simulink model "tg9"  (R2022a)
settings: Solver=ode15s  StartTime=0.0  StopTime=10  MaxStep=0.01  RelTol=1e-3
InitFcn:
  | mecha_param2
  | control_param0
values from neighbouring files (symbols this model uses):
  b0 = 0    [sim_IMMC.m]
  b1 = 1    [sim_IMMC.m]
  back0 = 0    [sim_IMMC.m]
  back1 = 0    [sim_IMMC.m]
  boff = 0    [sim_IMMC.m]
  bon = 0    [sim_IMMC.m]
  c = 0.05    [mecha_param2.m]
  c_jointstop = 0.3 / (pi/180)    (= 17.1887338539)    [mecha_param2.m]
  calctalus = sqrt((L_foot - (DJ1x_foot))^2 + (H_foot-r_cs)^2)    [mecha_param2.m]
  calctoes = sqrt((H_foot-r_cs)^2 + (DJ1x_foot)^2)    [mecha_param2.m]
  corrD = 0.001    [control_param0.m]
  DG_HAT = 0.35    [mecha_param2.m]
  DG_thigh = 0.28    [mecha_param2.m]
  DJ1x_foot = 0.16-r_cs    (= 0.135)    [mecha_param2.m]
  eref = 0.04    [mecha_param2.m]
  FmaxBFSH = 350    [mecha_param2.m]
  FmaxGAS = 1500    [mecha_param2.m]
  FmaxGLU = 1500    [mecha_param2.m]
  FmaxHAM = 3000    [mecha_param2.m]
  FmaxHFL = 2000    [mecha_param2.m]
  FmaxRF = 1200    [mecha_param2.m]
  FmaxSOL = 4000    [mecha_param2.m]
  FmaxTA = 800    [mecha_param2.m]
  FmaxVAS = 6000    [mecha_param2.m]
  g = 9.81    [mecha_param2.m]
  g0 = 0    [sim_IMMC.m]
  g1 = 0    [sim_IMMC.m]
  H_foot = 0.08    [mecha_param2.m]
  In_HAT = 3    [mecha_param2.m]
  In_shank = 0.05    [mecha_param2.m]
  In_thigh = 0.15    [mecha_param2.m]
  K = 5    [mecha_param2.m]
  knee_thigh = [0 0 -(L_thigh/2)]    [mecha_param2.m]
  Kpress = m_HAT * g / DeltaThRef    (= 104967)    [mecha_param2.m]
  L_foot = 0.2    [mecha_param2.m]
  L_HAT = 0.8    [mecha_param2.m]
  L_shank = 0.46    [mecha_param2.m]
  L_thigh = 0.46    [mecha_param2.m]
  LoHAM = table2array(mt('LoHAM', 1))    [control_param0.m]
  LoHFL = table2array(mt('LoHFL', 1))    [control_param0.m]
  longD = longD - corrD    (= 0.019)    [control_param0.m]
  loptBFSH = 0.12    [mecha_param2.m]
  loptGAS = 0.05    [mecha_param2.m]
  loptGLU = 0.11    [mecha_param2.m]
  loptHAM = 0.10    (= 0.1)    [mecha_param2.m]
  loptHFL = 0.11    [mecha_param2.m]
  loptRF = 0.08    [mecha_param2.m]
  loptSOL = 0.04    [mecha_param2.m]
  loptTA = 0.06    [mecha_param2.m]
  loptVAS = 0.08    [mecha_param2.m]
  LoTA = table2array(mt('LoTA', 1))    [control_param0.m]
  lslackBFSH = 0.10    (= 0.1)    [mecha_param2.m]
  lslackGAS = 0.40    (= 0.4)    [mecha_param2.m]
  lslackGLU = 0.13    [mecha_param2.m]
  lslackHAM = 0.31    [mecha_param2.m]
  lslackHFL = 0.10    (= 0.1)    [mecha_param2.m]
  lslackRF = 0.35    [mecha_param2.m]
  lslackSOL = 0.26    [mecha_param2.m]
  lslackTA = 0.24    [mecha_param2.m]
  lslackVAS = 0.23    [mecha_param2.m]
  m_HAT = 53.5    [mecha_param2.m]
  m_shank = 3.5    [mecha_param2.m]
  m_thigh = 8.5    [mecha_param2.m]
  midD = midD - corrD    (= 0.009)    [control_param0.m]
  N = 1.5    [mecha_param2.m]
  nonoff = 0    [control_param0.m]
  phi_a_low = (70) * (pi / 180)    (= 1.2217304764)    [mecha_param2.m]
  phi_a_up = (130) * (pi / 180)    (= 2.26892802759)    [mecha_param2.m]
  phi_dl = 180    [mecha_param2.m]
  phi_h = 230 * (pi / 180)    (= 4.01425727959)    [mecha_param2.m]
  phi_k = 175 * (pi / 180)    (= 3.05432619099)    [mecha_param2.m]
  phictoes = asind((DJ1y_foot-r_cs)/calctoes)    [mecha_param2.m]
  phimaxGASa = 100*pi/180    (= 1.74532925199)    [mecha_param2.m]
  phimaxGASk = 140*pi/180    (= 2.44346095279)    [mecha_param2.m]
  phimaxRFk = 165*pi/180    (= 2.87979326579)    [mecha_param2.m]
  phimaxSOL = 100*pi/180    (= 1.74532925199)    [mecha_param2.m]
  phimaxTA = 80*pi/180    (= 1.3962634016)    [mecha_param2.m]
  phimaxVAS = 165*pi/180    (= 2.87979326579)    [mecha_param2.m]
  phirefBFSH = 160*pi/180    (= 2.79252680319)    [mecha_param2.m]
  phirefGASa = 80*pi/180    (= 1.3962634016)    [mecha_param2.m]
  phirefGASk = 165*pi/180    (= 2.87979326579)    [mecha_param2.m]
  phirefGLU = 120*pi/180    (= 2.09439510239)    [mecha_param2.m]
  phirefHAMh = 150*pi/180    (= 2.61799387799)    [mecha_param2.m]
  phirefHAMk = 180*pi/180    (= 3.14159265359)    [mecha_param2.m]
  phirefHFL = 160*pi/180    (= 2.79252680319)    [mecha_param2.m]
  phirefRFh = 170*pi/180    (= 2.96705972839)    [mecha_param2.m]
  phirefRFk = 125*pi/180    (= 2.18166156499)    [mecha_param2.m]
  phirefSOL = 90*pi/180    (= 1.57079632679)    [mecha_param2.m]
  phirefTA = 110*pi/180    (= 1.91986217719)    [mecha_param2.m]
  phirefVAS = 120*pi/180    (= 2.09439510239)    [mecha_param2.m]
  phiScaleGASa = acos(rGASamin/rGASamax)/(phiminGASa-phimaxGASa)    [mecha_param2.m]
  phiScaleGASk = acos(rGASkmin/rGASkmax)/(phiminGASk-phimaxGASk)    [mecha_param2.m]
  phiScaleRFk = acos(rRFkmin/rRFkmax)/(phiminRFk-phimaxRFk)    [mecha_param2.m]
  phiScaleSOL = acos(rSOLmin/rSOLmax)/(phiminSOL-phimaxSOL)    [mecha_param2.m]
  phiScaleTA = acos(rTAmin/rTAmax)/(phiminTA-phimaxTA)    [mecha_param2.m]
  phiScaleVAS = acos(rVASmin/rVASmax)/(phiminVAS-phimaxVAS)    [mecha_param2.m]
  r1 = 0    [sim_IMMC.m]
  r_cs = 0.025    [mecha_param2.m]
  rBFSH = 0.04    [mecha_param2.m]
  rGASamax = 0.06    [mecha_param2.m]
  rGASkmax = 0.05    [mecha_param2.m]
  rGLU = 0.08    [mecha_param2.m]
  rHAMh = 0.08    [mecha_param2.m]
  rHAMk = 0.05    [mecha_param2.m]
  rHFL = 0.08    [mecha_param2.m]
  rhoBFSH = 0.7    [mecha_param2.m]
  rhoGASa = 0.7    [mecha_param2.m]
  rhoGASk = 0.7    [mecha_param2.m]
  rhoGLU = 0.5    [mecha_param2.m]
  rhoHAMh = 0.5    [mecha_param2.m]
  rhoHAMk = 0.5    [mecha_param2.m]
  rhoHFL = 0.5    [mecha_param2.m]
  rhoRFh = 0.3    [mecha_param2.m]
  rhoRFk = 0.5    [mecha_param2.m]
  rhoSOL = 0.5    [mecha_param2.m]
  rhoTA = 0.7    [mecha_param2.m]
  rhoVAS = 0.6    [mecha_param2.m]
  rRFh = 0.08    [mecha_param2.m]
  rRFkmax = 0.06    [mecha_param2.m]
  rSOLmax = 0.06    [mecha_param2.m]
  ... (+25 more)
undefined symbols (not defined in the file or in its folder): beta11, beta12, beta13, beta14, beta15, beta16, beta21, beta22, beta23, beta24, beta25, beta26, beta31, beta32, beta33, beta34, beta35, beta36, beta41, beta42, beta43, beta44, beta45, beta46, beta51, beta52, beta53, beta54, beta55, beta56, betab1, betab2, betab3, betab4, betab5, betab6, betap11, betap12, betap13, betap14, betap15, betap16, betap21, betap22, betap23, betap24, betap25, betap26, betap31, betap32, betap33, betap34, betap35, betap36, betap41, betap42, betap43, betap44, betap45, betap46 ... (+102)
libraries: sm_lib x89, simulink x72, nesl_utility x58, simulink_extras x18
(part 2 of 12)

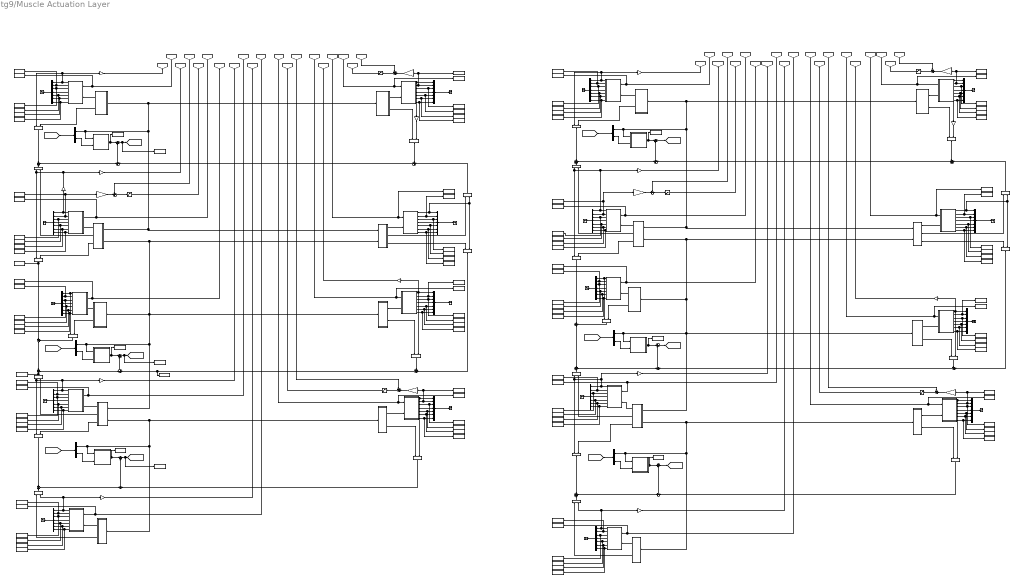
== system tg9/Muscle Actuation Layer ==
  note: L-Lo
  note: Left Hip Joint Mechanics Layer Interface
  note: Right leg - muscular/sensor layer
  note: Muscle Actuator Layer
  note: Left leg - muscular/sensor layer
  note: Left Knee Joint Mechanics Layer Interface
  note: Left Ankle Joint Mechanics Layer Interface
  note: Right Hip Joint Mechanics Layer Interface
  note: Right Knee Joint Mechanics Layer Interface
  note: Right Ankle Joint Mechanics Layer Interface
  note: L-Lo
  note: L-Lo
  note: L-Lo
  note: L-Lo
  note: L-Lo
  Demux{3..8} (6 alike) : Demux  Outputs=2
  Gain : Gain  Gain=1/loptHAM
  Gain1 : Gain  Gain=1/loptHFL
  Gain2 : Gain  Gain=1/loptTA
  Gain3 : Gain  Gain=1/loptHAM
  Gain4 : Gain  Gain=1/loptHFL
  Gain5 : Gain  Gain=1/loptTA
  Gain6 : Gain
  Gain7 : Gain
  Gain9 : Gain
  L Ankle Joint Limit : Subsystem
  L BFSH : Subsystem
  L BFSH Link1 : Subsystem
  L BFSH Link2 : Subsystem
  L GAS : Subsystem
  L GAS Golgi Tendon Organ : Gain
  L GAS Link1 : Subsystem
  L GAS Link2 : Subsystem
  L GLU : Subsystem
  L GLU Golgi Tendon Organ : Gain
  L GLU Link : Subsystem
  L GLU Link1 : Subsystem
  L HAM : Subsystem
  L HAM Golgi Tendon Organ : Gain
  L HAM Link1 : Subsystem
  L HAM Link2 : Subsystem
  L HFL : Subsystem
  L HFL Link1 : Subsystem
  L HFL Link2 : Subsystem
  L Hip Joint Limits : Subsystem
  L Knee Joint Limits : Subsystem
  L RF : Subsystem
  L RF Link1 : Subsystem
  L RF Link2 : Subsystem
  L SOL : Subsystem
  L SOL Golgi Tendon Organ : Gain
  L SOL Link1 : Subsystem
  L SOL Link2 : Subsystem
  L TA : Subsystem
  L TA Link1 : Subsystem
  L TA Link2 : Subsystem
  L VAS : Subsystem
  L VAS Golgi Tendon Organ : Gain
  L VAS Link1 : Subsystem
  L VAS Link2 : Subsystem
  Mux{,1..17} (18 alike) : Mux  Inputs=7
  Product{,1..23} (24 alike) : Product
  R Ankle Joint Limit : Subsystem
  R BFSH : Subsystem
  R GAS : Subsystem
  R GAS Golgi Tendon Organ : Gain
  R GLU : Subsystem
  R GLU Golgi Tendon Organ : Gain
  R HAM Golgi Tendon Organ : Gain
  R HAM1 : Subsystem
  R HFL : Subsystem
  R Hip Joint Limits : Subsystem
  R Knee Joint Limits : Subsystem
  R RF : Subsystem
  R SOL : Subsystem
  R SOL Golgi Tendon Organ : Gain
  R TA : Subsystem
  R VAS : Subsystem
  R VAS Golgi Tendon Organ : Gain
  Saturation{,1..5} (6 alike) : Saturate  UpperLimit=inf  LowerLimit=0  ZeroCross=off
  Sum{,3,6,12,17,20,24,27} (8 alike) : Sum  Inputs=|++
  Sum{1,7,13,21} (4 alike) : Sum  Inputs=+|-
  Sum{9..11,14..15,23} (6 alike) : Sum  Inputs=-+|
  Sum{2,5,8,16,19,22} (6 alike) : Sum  Inputs=+|+
  Sum18 : Sum  Inputs=-|+
  Sum{25..26,28..29} (4 alike) : Sum  Inputs=++|
  Sum4 : Sum  Inputs=-|+
  Terminator{,1..17} (18 alike) : Terminator
  To Workspace : ToWorkspace  VariableName=RHFL_ACT  SampleTime=-1
  To Workspace1 : ToWorkspace  VariableName=RHFL_STIM  SampleTime=-1
  To Workspace10 : ToWorkspace  VariableName=RVAS_STIM  SampleTime=-1
  To Workspace100 : ToWorkspace  VariableName=LRF_FISO  SampleTime=-1
  To Workspace101 : ToWorkspace  VariableName=LRF_LCE  SampleTime=-1
  To Workspace102 : ToWorkspace  VariableName=LBFSH_STIM  SampleTime=-1
  To Workspace103 : ToWorkspace  VariableName=LBFSH_LCE  SampleTime=-1
  To Workspace104 : ToWorkspace  VariableName=LBFSH_ACT  SampleTime=-1
  To Workspace105 : ToWorkspace  VariableName=LBFSH_VCE  SampleTime=-1
  To Workspace106 : ToWorkspace  VariableName=LBFSH_FCE  SampleTime=-1
  To Workspace107 : ToWorkspace  VariableName=LBFSH_FISO  SampleTime=-1
  To Workspace108 : ToWorkspace  VariableName=RBFSH_STIM  SampleTime=-1
  To Workspace109 : ToWorkspace  VariableName=RBFSH_LCE  SampleTime=-1
  To Workspace11 : ToWorkspace  VariableName=RVAS_LCE  SampleTime=-1
  To Workspace110 : ToWorkspace  VariableName=RBFSH_ACT  SampleTime=-1
  To Workspace111 : ToWorkspace  VariableName=RBFSH_VCE  SampleTime=-1
  To Workspace112 : ToWorkspace  VariableName=RBFSH_FCE  SampleTime=-1
  To Workspace113 : ToWorkspace  VariableName=RBFSH_FISO  SampleTime=-1
  To Workspace114 : ToWorkspace  VariableName=RRF_FISO  SampleTime=-1
  To Workspace115 : ToWorkspace  VariableName=RRF_LCE  SampleTime=-1
  To Workspace116 : ToWorkspace  VariableName=RRF_ACT  SampleTime=-1
  To Workspace117 : ToWorkspace  VariableName=RRF_STIM  SampleTime=-1
  To Workspace118 : ToWorkspace  VariableName=RRF_VCE  SampleTime=-1
  To Workspace119 : ToWorkspace  VariableName=RRF_FCE  SampleTime=-1
  To Workspace12 : ToWorkspace  VariableName=RTA_STIM  SampleTime=-1
  To Workspace13 : ToWorkspace  VariableName=RTA_LCE  SampleTime=-1
  To Workspace14 : ToWorkspace  VariableName=RTA_ACT  SampleTime=-1
  To Workspace15 : ToWorkspace  VariableName=RTA_VCE  SampleTime=-1
  To Workspace16 : ToWorkspace  VariableName=RTA_FCE  SampleTime=-1
  To Workspace17 : ToWorkspace  VariableName=RTA_FISO  SampleTime=-1
  To Workspace18 : ToWorkspace  VariableName=RGAS_STIM  SampleTime=-1
  To Workspace19 : ToWorkspace  VariableName=RGAS_LCE  SampleTime=-1
  To Workspace2 : ToWorkspace  VariableName=RHFL_VCE  SampleTime=-1
  To Workspace20 : ToWorkspace  VariableName=RGAS_ACT  SampleTime=-1
  To Workspace21 : ToWorkspace  VariableName=RGAS_VCE  SampleTime=-1
  To Workspace22 : ToWorkspace  VariableName=RGAS_FCE  SampleTime=-1
  To Workspace23 : ToWorkspace  VariableName=RGAS_FISO  SampleTime=-1
  To Workspace24 : ToWorkspace  VariableName=RSOL_STIM  SampleTime=-1
  To Workspace25 : ToWorkspace  VariableName=RSOL_LCE  SampleTime=-1
  To Workspace26 : ToWorkspace  VariableName=RSOL_ACT  SampleTime=-1
  To Workspace27 : ToWorkspace  VariableName=RSOL_VCE  SampleTime=-1
  To Workspace28 : ToWorkspace  VariableName=RSOL_FCE  SampleTime=-1
  To Workspace29 : ToWorkspace  VariableName=RSOL_FISO  SampleTime=-1
  To Workspace3 : ToWorkspace  VariableName=RHFL_FCE  SampleTime=-1
  To Workspace30 : ToWorkspace  VariableName=RHAM_STIM  SampleTime=-1
  To Workspace31 : ToWorkspace  VariableName=RHAM_LCE  SampleTime=-1
  To Workspace32 : ToWorkspace  VariableName=RHAM_ACT  SampleTime=-1
  To Workspace33 : ToWorkspace  VariableName=RHAM_VCE  SampleTime=-1
  To Workspace34 : ToWorkspace  VariableName=RHAM_FCE  SampleTime=-1
  To Workspace35 : ToWorkspace  VariableName=RHAM_FISO  SampleTime=-1
  To Workspace36 : ToWorkspace  VariableName=RGLU_STIM  SampleTime=-1
  To Workspace37 : ToWorkspace  VariableName=RGLU_LCE  SampleTime=-1
  To Workspace38 : ToWorkspace  VariableName=RGLU_ACT  SampleTime=-1
  To Workspace39 : ToWorkspace  VariableName=RGLU_VCE  SampleTime=-1
  To Workspace4 : ToWorkspace  VariableName=RHFL_FISO  SampleTime=-1
  To Workspace40 : ToWorkspace  VariableName=RGLU_FCE  SampleTime=-1
  To Workspace41 : ToWorkspace  VariableName=RGLU_FISO  SampleTime=-1
  To Workspace42 : ToWorkspace  VariableName=LHFL_ACT  SampleTime=-1
  To Workspace43 : ToWorkspace  VariableName=LHFL_STIM  SampleTime=-1
  To Workspace44 : ToWorkspace  VariableName=LHFL_VCE  SampleTime=-1
  To Workspace45 : ToWorkspace  VariableName=LHFL_FCE  SampleTime=-1
  To Workspace46 : ToWorkspace  VariableName=LHFL_FISO  SampleTime=-1
  To Workspace47 : ToWorkspace  VariableName=LHFL_LCE  SampleTime=-1
  To Workspace48 : ToWorkspace  VariableName=LVAS_ACT  SampleTime=-1
  To Workspace49 : ToWorkspace  VariableName=LVAS_STIM  SampleTime=-1
  To Workspace5 : ToWorkspace  VariableName=RHFL_LCE  SampleTime=-1
  To Workspace50 : ToWorkspace  VariableName=LVAS_VCE  SampleTime=-1
  To Workspace51 : ToWorkspace  VariableName=LVAS_FCE  SampleTime=-1
  To Workspace52 : ToWorkspace  VariableName=LVAS_FISO  SampleTime=-1
  To Workspace53 : ToWorkspace  VariableName=LVAS_LCE  SampleTime=-1
  To Workspace54 : ToWorkspace  VariableName=LTA_ACT  SampleTime=-1
  To Workspace55 : ToWorkspace  VariableName=LTA_STIM  SampleTime=-1
  To Workspace56 : ToWorkspace  VariableName=LTA_VCE  SampleTime=-1
  To Workspace57 : ToWorkspace  VariableName=LTA_FCE  SampleTime=-1
  To Workspace58 : ToWorkspace  VariableName=LTA_FISO  SampleTime=-1
  To Workspace59 : ToWorkspace  VariableName=LTA_LCE  SampleTime=-1
  To Workspace6 : ToWorkspace  VariableName=RVAS_ACT  SampleTime=-1
  To Workspace60 : ToWorkspace  VariableName=LGLU_STIM  SampleTime=-1
  To Workspace61 : ToWorkspace  VariableName=LGLU_LCE  SampleTime=-1
  To Workspace62 : ToWorkspace  VariableName=LGLU_ACT  SampleTime=-1
  To Workspace63 : ToWorkspace  VariableName=LGLU_VCE  SampleTime=-1
  To Workspace64 : ToWorkspace  VariableName=LGLU_FCE  SampleTime=-1
  To Workspace65 : ToWorkspace  VariableName=LGLU_FISO  SampleTime=-1
  To Workspace66 : ToWorkspace  VariableName=LHAM_STIM  SampleTime=-1
  To Workspace67 : ToWorkspace  VariableName=LHAM_LCE  SampleTime=-1
  To Workspace68 : ToWorkspace  VariableName=LHAM_ACT  SampleTime=-1
  To Workspace69 : ToWorkspace  VariableName=LHAM_VCE  SampleTime=-1
  To Workspace7 : ToWorkspace  VariableName=RVAS_VCE  SampleTime=-1
  To Workspace70 : ToWorkspace  VariableName=LHAM_FCE  SampleTime=-1
  To Workspace71 : ToWorkspace  VariableName=LHAM_FISO  SampleTime=-1
  To Workspace72 : ToWorkspace  VariableName=LGAS_STIM  SampleTime=-1
  To Workspace73 : ToWorkspace  VariableName=LGAS_LCE  SampleTime=-1
  To Workspace74 : ToWorkspace  VariableName=LGAS_ACT  SampleTime=-1
  To Workspace75 : ToWorkspace  VariableName=LGAS_VCE  SampleTime=-1
  To Workspace76 : ToWorkspace  VariableName=LGAS_FCE  SampleTime=-1
  To Workspace77 : ToWorkspace  VariableName=LGAS_FISO  SampleTime=-1
  To Workspace78 : ToWorkspace  VariableName=LSOL_STIM  SampleTime=-1
  To Workspace79 : ToWorkspace  VariableName=LSOL_LCE  SampleTime=-1
  To Workspace8 : ToWorkspace  VariableName=RVAS_FCE  SampleTime=-1
  To Workspace80 : ToWorkspace  VariableName=LSOL_ACT  SampleTime=-1
  To Workspace81 : ToWorkspace  VariableName=LSOL_VCE  SampleTime=-1
  To Workspace82 : ToWorkspace  VariableName=LSOL_FCE  SampleTime=-1
  To Workspace83 : ToWorkspace  VariableName=LSOL_FISO  SampleTime=-1
  To Workspace84 : ToWorkspace  VariableName=painLhip  SampleTime=-1
  To Workspace85 : ToWorkspace  VariableName=painLknee  SampleTime=-1
  To Workspace86 : ToWorkspace  VariableName=painLankle  SampleTime=-1
  To Workspace87 : ToWorkspace  VariableName=painRankle  SampleTime=-1
  To Workspace88 : ToWorkspace  VariableName=painRknee  SampleTime=-1
  To Workspace89 : ToWorkspace  VariableName=painRhip  SampleTime=-1
  To Workspace9 : ToWorkspace  VariableName=RVAS_FISO  SampleTime=-1
  To Workspace90 : ToWorkspace  VariableName=LhipT  SampleTime=-1
  To Workspace91 : ToWorkspace  VariableName=LkneeT  SampleTime=-1
  To Workspace92 : ToWorkspace  VariableName=LankleT  SampleTime=-1
  To Workspace93 : ToWorkspace  VariableName=VASf  SampleTime=-1
  To Workspace94 : ToWorkspace  VariableName=HAMf  SampleTime=-1
  To Workspace95 : ToWorkspace  VariableName=GASf  SampleTime=-1
  To Workspace96 : ToWorkspace  VariableName=LRF_ACT  SampleTime=-1
  To Workspace97 : ToWorkspace  VariableName=LRF_STIM  SampleTime=-1
  To Workspace98 : ToWorkspace  VariableName=LRF_VCE  SampleTime=-1
  To Workspace99 : ToWorkspace  VariableName=LRF_FCE  SampleTime=-1
  tag scope: LGASgolgi=global, LGLUgolgi=global, LHAMgolgi=global, LHAMspindle=global, LHFLspindle=global, LSOLgolgi=global, LTAspindle=global, LVASgolgi=global, LankleM=global, LhipM=global, LkneeM=global, RGASgolgi=global, RGLUgolgi=global, RHAMgolgi=global, RHAMspindle=global, RHFLspindle=global, RSOLgolgi=global, RTAspindle=global, RVASgolgi=global, RankleM=global, RhipM=global, RkneeM=global
  wires:
  Demux3/1 -> L Hip Joint Limits/1(phi hip [rad]), L GLU Link/1(phi34 [rad]), L HFL Link1/1(phi34 [rad]), L HAM Link2/1(phi34 [rad]), L RF Link1/1(phi34 [rad])
  Demux3/2 -> L Hip Joint Limits/2(dphi hip [rad/s])
  [LHipBMLMAL] -> Demux3/1
  Demux4/1 -> L GAS Link1/1(phi23 [rad]), L BFSH Link1/1(phi23 [rad]), L VAS Link1/1(phi23 [rad]), L HAM Link2/2(phi23 [rad]), L RF Link1/2(phi23 [rad]), L Knee Joint Limits/1(phi [rad])
  [LKneeBMLMAL] -> Demux4/1
  Demux4/2 -> L Knee Joint Limits/2(dphi [rad/s])
  Demux5/2 -> L Ankle Joint Limit/2(dphi [rad/s])
  Demux5/1 -> L SOL Link1/1(phi12 [rad]), L GAS Link1/2(phi12 [rad]), L TA Link1/1(phi12 [rad]), L Ankle Joint Limit/1(phi [rad])
  [LAnkleBMLMAL] -> Demux5/1
  L Hip Joint Limits/1(M_stop [Nm]) -> To Workspace84/1, Sum/1
  Sum/1 -> To Workspace90/1, [LhipM]
  Sum1/1 -> Sum/2
  Sum2/1 -> Sum1/1
  Sum3/1 -> To Workspace91/1, [LkneeM]
  Sum4/1 -> Sum3/2
  Sum5/1 -> Sum4/1
  Sum6/1 -> To Workspace92/1, [LankleM]
  L Ankle Joint Limit/1(M_stop [Nm]) -> To Workspace86/1, Sum6/1
  Sum8/1 -> Sum7/1
  Sum7/1 -> Sum6/2
  [LGLUstim] -> To Workspace60/1, L GLU/1(STIM)
  L GLU Link/1(lmtu [m]) -> L GLU/2(lmtu [m])
  L GLU/1(Fmtc) -> Mux/1, L GLU Golgi Tendon Organ/1, Product/1
  L GLU/2(Lce) -> To Workspace61/1, Mux/2
  L GLU/4(lse) -> Mux/4
  L GLU/5(A) -> To Workspace62/1, Mux/5
  Mux/1 -> Terminator/1
  Mux1/1 -> Terminator7/1
  L HFL/4(lse) -> Mux1/4
  L HFL/2(Lce) -> Mux1/2, To Workspace47/1, Gain1/1
  L HFL/5(A) -> Mux1/5, To Workspace42/1
  L HFL/1(Fmtc) -> Gain6/1, Mux1/1
  L HFL Link1/1(lmtu [m]) -> L HFL/2(lmtu [m])
  L HFL/3(Vce) -> To Workspace44/1, Mux1/3
  [LHFLstim] -> To Workspace43/1, L HFL/1(STIM)
  L VAS/4(lse) -> Mux2/4
  L VAS/1(Fmtc) -> Mux2/1, Product7/2, L VAS Golgi Tendon Organ/1
  L VAS/2(Lce) -> To Workspace53/1, Mux2/2
  L VAS/5(A) -> To Workspace48/1, Mux2/5
  [LVASstim] -> To Workspace49/1, L VAS/1(STIM)
  Mux2/1 -> Terminator1/1
  L HAM/4(lse) -> Mux3/4
  L HAM/1(Fmtc) -> Mux3/1, Gain9/1
  L HAM/2(Lce) -> Mux3/2, Gain/1, To Workspace67/1
  L HAM/5(A) -> Mux3/5, To Workspace68/1
  [LHAMstim] -> To Workspace66/1, L HAM/1(STIM)
  L HAM/3(Vce) -> To Workspace69/1, Mux3/3
  Mux3/1 -> Terminator8/1
  L HAM Link2/1(lmtu [m]) -> L HAM/2(lmtu [m])
  L VAS Link1/1(lmtu [m]) -> L VAS/2(lmtu [m])
  L GAS/4(lse) -> Mux4/4
  L GAS/1(Fmtc) -> Mux4/1, L GAS Golgi Tendon Organ/1, Product4/1, Product3/1
  L GAS/2(Lce) -> To Workspace73/1, Mux4/2
  L GAS/5(A) -> To Workspace74/1, Mux4/5
  L GAS/3(Vce) -> To Workspace75/1, Mux4/3
  Mux4/1 -> Terminator2/1
  L GAS Link1/1(lmtu [m]) -> L GAS/2(lmtu [m])
  L TA Link1/1(lmtc [m]) -> L TA/2(lmtu [m])
  L TA/4(lse) -> Mux5/4
  L TA/1(Fmtc) -> Product6/2, Mux5/1
  L TA/2(Lce) -> Mux5/2, Gain2/1, To Workspace59/1
  L TA/5(A) -> To Workspace54/1, Mux5/5
  [LTAstim] -> To Workspace55/1, L TA/1(STIM)
  L TA/3(Vce) -> To Workspace56/1, Mux5/3
  Mux5/1 -> Terminator3/1
  L SOL/4(lse) -> Mux6/4
  L SOL/1(Fmtc) -> Mux6/1, L SOL Golgi Tendon Organ/1, Product5/2
  L SOL/2(Lce) -> To Workspace79/1, Mux6/2
  L SOL/5(A) -> To Workspace80/1, Mux6/5
  L SOL/3(Vce) -> To Workspace81/1, Mux6/3
  Mux6/1 -> Terminator4/1
  L SOL Link1/1(lmtc [m]) -> L SOL/2(lmtu [m])
  L GLU Link/2(lever [m]) -> Product/2
  Product/1 -> Sum2/1
  Product1/1 -> Sum2/2
  L HAM Link2/2(lever34 [m]) -> Product1/2
  L HAM Link2/3(lever23 [m]) -> Product2/2
  Sum24/1 -> Sum5/1
  Product3/1 -> To Workspace95/1, Sum5/2
  L GAS Link1/2(lever23 [m]) -> Product3/2
  L GAS Link1/3(lever12 [m]) -> Product4/2
  Product4/1 -> Sum8/1
  Product5/1 -> Sum8/2
  L SOL Link1/2(lever [m]) -> Product5/1
  L TA Link1/2(lever [m]) -> Product6/1
  Product6/1 -> Sum7/2
  Sum25/1 -> To Workspace93/1, Sum4/2
  L VAS Link1/2(lever [m]) -> Product7/1
  L VAS/3(Vce) -> To Workspace50/1, Mux2/3
  L HFL Link1/2(lever [m]) -> Product8/1
  Sum26/1 -> Sum1/2
  L GLU Golgi Tendon Organ/1 -> [LGLUgolgi]
  L HAM Golgi Tendon Organ/1 -> [LHAMgolgi]
  L SOL Golgi Tendon Organ/1 -> [LSOLgolgi]
  L GAS Golgi Tendon Organ/1 -> [LGASgolgi]
  Gain/1 -> Sum9/2
  Sum9/1 -> Saturation/1
  Gain1/1 -> Sum10/2
  Sum10/1 -> Saturation1/1
  Gain2/1 -> Sum11/2
  Sum11/1 -> Saturation2/1
  L VAS Golgi Tendon Organ/1 -> [LVASgolgi]
  Saturation/1 -> [LHAMspindle]
  [LyHAM] -> Sum9/1
  [LGASstim] -> To Workspace72/1, L GAS/1(STIM)
  [LSOLstim] -> To Workspace78/1, L SOL/1(STIM)
  [LyTA] -> Sum11/1
  [LyHFL] -> Sum10/1
  Saturation2/1 -> [LTAspindle]
  Saturation1/1 -> [LHFLspindle]
  Demux8/1 -> R Ankle Joint Limit/1(phi [rad]), L SOL Link2/1(phi12 [rad]), L TA Link2/1(phi12 [rad]), L GAS Link2/2(phi12 [rad])
  Saturation4/1 -> [RHFLspindle]
  Product11/1 -> Sum27/1
  Mux7/1 -> Terminator5/1
  L GLU Link1/2(lever [m]) -> Product9/2
  L SOL Link2/2(lever [m]) -> Product14/1
  Mux9/1 -> Terminator6/1
  Sum17/1 -> [RkneeM]
  Gain4/1 -> Sum14/2
  R VAS/1(Fmtc) -> R VAS Golgi Tendon Organ/1, Product16/2, Mux9/1
  L TA Link2/1(lmtc [m]) -> R TA/2(lmtu [m])
  R GAS Golgi Tendon Organ/1 -> [RGASgolgi]
  R VAS/3(Vce) -> To Workspace7/1, Mux9/3
  Saturation5/1 -> [RTAspindle]
  R SOL/4(lse) -> Mux13/4
  R VAS Golgi Tendon Organ/1 -> [RVASgolgi]
  [RyHFL] -> Sum14/1
  Gain3/1 -> Sum23/2
  Sum16/1 -> Sum13/1
  [RGASstim] -> R GAS/1(STIM), To Workspace18/1
  Sum18/1 -> Sum17/2
  R TA/2(Lce) -> Gain5/1, To Workspace13/1, Mux12/2
  Sum15/1 -> Saturation5/1
  R SOL Golgi Tendon Organ/1 -> [RSOLgolgi]
  L HAM Link1/2(lever34 [m]) -> Product10/2
  Sum28/1 -> Sum18/2
  [RyTA] -> Sum15/1
  [RyHAM] -> Sum23/1
  R Ankle Joint Limit/1(M_stop [Nm]) -> To Workspace87/1, Sum20/1
  R VAS/2(Lce) -> Mux9/2, To Workspace11/1
  R GLU Golgi Tendon Organ/1 -> [RGLUgolgi]
  L HFL Link2/2(lever [m]) -> Product17/1
  R HFL/3(Vce [m/s]) -> To Workspace2/1, Mux8/3
  Mux11/1 -> Terminator9/1
  R VAS/5(A) -> To Workspace6/1, Mux9/5
  Saturation3/1 -> [RHAMspindle]
  Sum13/1 -> Sum12/2
  Sum14/1 -> Saturation4/1
  Sum23/1 -> Saturation3/1
  Sum29/1 -> Sum13/2
  Sum20/1 -> [RankleM]
  Product13/1 -> Sum22/1
  R HAM1/3(Vce) -> Mux10/3, To Workspace33/1
  Product12/1 -> Sum19/2
  L HAM Link1/3(lever23 [m]) -> Product11/2
  L VAS Link2/1(lmtu [m]) -> R VAS/2(lmtu [m])
  R GAS/5(A) -> To Workspace20/1, Mux11/5
  L GAS Link2/2(lever23 [m]) -> Product12/2
  Product14/1 -> Sum22/2
  Product15/1 -> Sum21/2
  L HFL Link2/1(lmtu [m]) -> R HFL/2(lmtu [m])
  L GAS Link2/3(lever12 [m]) -> Product13/2
  L TA Link2/2(lever [m]) -> Product15/1
  R GAS/4(lse) -> Mux11/4
  Product10/1 -> Sum16/2
  [RAnkleBMLMAL] -> Demux8/1
  Product9/1 -> Sum16/1
  Mux12/1 -> Terminator10/1
  L SOL Link2/1(lmtc [m]) -> R SOL/2(lmtu [m])
  Mux13/1 -> Terminator11/1
  R GAS/1(Fmtc) -> Mux11/1, R GAS Golgi Tendon Organ/1, Product12/1, Product13/1
  R GAS/2(Lce) -> To Workspace19/1, Mux11/2
  R VAS/4(lse) -> Mux9/4
  [RHAMstim] -> To Workspace30/1, R HAM1/1(STIM)
  [RHFLstim] -> To Workspace1/1, R HFL/1(STIM)
  R HAM1/2(Lce) -> Mux10/2, To Workspace31/1, Gain3/1
  [RTAstim] -> To Workspace12/1, R TA/1(STIM)
  L GAS Link2/1(lmtu [m]) -> R GAS/2(lmtu [m])
  R TA/3(Vce) -> To Workspace15/1, Mux12/3
  R HAM1/5(A) -> To Workspace32/1, Mux10/5
  R TA/5(A) -> To Workspace14/1, Mux12/5
  R TA/4(lse) -> Mux12/4
  Sum21/1 -> Sum20/2
  R HFL/4(lse [m]) -> Mux8/4
  R HAM1/4(lse) -> Mux10/4
  R GLU/4(lse) -> Mux7/4
  R GLU/3(Vce) -> To Workspace39/1, Mux7/3
  [RGLUstim] -> To Workspace36/1, R GLU/1(STIM)
  L VAS Link2/2(lever [m]) -> Product16/1
  Mux10/1 -> Terminator13/1
  Mux8/1 -> Terminator12/1
  Gain5/1 -> Sum15/2
  R HAM Golgi Tendon Organ/1 -> [RHAMgolgi]
  R GLU/5(A) -> To Workspace38/1, Mux7/5
  R GAS/3(Vce) -> To Workspace21/1, Mux11/3
  [RHipBMLMAL] -> Demux6/1
  R TA/1(Fmtc) -> Product15/2, Mux12/1
  R Knee Joint Limits/1(M_stop [Nm]) -> To Workspace88/1, Sum17/1
  [RKneeBMLMAL] -> Demux7/1
  [RSOLstim] -> To Workspace24/1, R SOL/1(STIM)
  R GLU/2(Lce) -> To Workspace37/1, Mux7/2
  R HFL/2(Lce [m]) -> To Workspace5/1, Gain4/1, Mux8/2
  Sum19/1 -> Sum18/1
  L HAM Link1/1(lmtu [m]) -> R HAM1/2(lmtu [m])
  L GLU Link1/1(lmtu [m]) -> R GLU/2(lmtu [m])
  R Hip Joint Limits/1(M_stop [Nm]) -> To Workspace89/1, Sum12/1
  Demux8/2 -> R Ankle Joint Limit/2(dphi [rad/s])
  R HAM1/1(Fmtc) -> Mux10/1, Product10/1, Product11/1, R HAM Golgi Tendon Organ/1
  R GLU/1(Fmtc) -> Mux7/1, R GLU Golgi Tendon Organ/1, Product9/1
  [RVASstim] -> To Workspace10/1, R VAS/1(STIM)
  Sum12/1 -> [RhipM]
  Demux7/2 -> R Knee Joint Limits/2(dphi [rad/s])
  Sum22/1 -> Sum21/1
  Demux6/2 -> R Hip Joint Limits/2(dphi [rad/s])
  Gain6/1 -> Product8/2
  Gain7/1 -> Product17/2
  Gain9/1 -> Product1/1, Product2/1, L HAM Golgi Tendon Organ/1
  R HFL/5(A) -> To Workspace/1, Mux8/5
  R HFL/1(Fmtc [N]) -> Gain7/1, Mux8/1
  R HFL/6(Fce [N]) -> To Workspace3/1, Mux8/6
  R HFL/7(fse [Fmax]) -> To Workspace4/1, Mux8/7
  R VAS/6(fce [Fmax]) -> To Workspace8/1, Mux9/6
  R VAS/7(fse [Fmax]) -> To Workspace9/1, Mux9/7
  R TA/6(fce [Fmax]) -> To Workspace16/1, Mux12/6
  R TA/7(fse [Fmax]) -> To Workspace17/1, Mux12/7
  R GAS/6(fce [Fmax]) -> To Workspace22/1, Mux11/6
  R GAS/7(fse [Fmax]) -> Mux11/7, To Workspace23/1
  R SOL/7("fse [Fmax}") -> To Workspace29/1, Mux13/7
  R SOL/6("fce [Fmax}") -> To Workspace28/1, Mux13/6
  R SOL/5(A) -> To Workspace26/1, Mux13/5
  R SOL/1(Fmtc) -> Mux13/1, R SOL Golgi Tendon Organ/1, Product14/2
  R SOL/3(Vce) -> To Workspace27/1, Mux13/3
  R SOL/2(Lce) -> Mux13/2, To Workspace25/1
  R HAM1/6(fce [Fmax]) -> To Workspace34/1, Mux10/6
  R HAM1/7(fse [Fmax]) -> To Workspace35/1, Mux10/7
  R GLU/6(fce [Fmax]) -> To Workspace40/1, Mux7/6
  R GLU/7(fse [Fmax]) -> To Workspace41/1, Mux7/7
  L SOL/6(fce [Fmax]) -> To Workspace82/1, Mux6/6
  L SOL/7("fse [Fmax}") -> To Workspace83/1, Mux6/7
  L GAS/6(fce [Fmax]) -> To Workspace76/1, Mux4/6
  L GAS/7("fse [Fmax}") -> To Workspace77/1, Mux4/7
  L HAM/6(fce [Fmax]) -> Mux3/6, To Workspace70/1
  L HAM/7("fse [Fmax}") -> To Workspace71/1, Mux3/7
  L GLU/6(fce [Fmax]) -> To Workspace64/1, Mux/6
  L GLU/7("fse [Fmax}") -> To Workspace65/1, Mux/7
  L HFL/6(fce [Fmax]) -> Mux1/6, To Workspace45/1
  L HFL/7("fse [Fmax}") -> To Workspace46/1, Mux1/7
  L VAS/6(fce [Fmax]) -> To Workspace51/1, Mux2/6
  L VAS/7("fse [Fmax}") -> To Workspace52/1, Mux2/7
  L TA/6(fce [Fmax]) -> To Workspace57/1, Mux5/6
  L TA/7("fse [Fmax}") -> To Workspace58/1, Mux5/7
  L GLU/3(Vce) -> Mux/3, To Workspace63/1
  L Knee Joint Limits/1(M_stop [Nm]) -> Sum3/1, To Workspace85/1
  L BFSH Link1/1(lmtu [m]) -> L BFSH/2(lmtu [m])
  Mux14/1 -> Terminator14/1
  L BFSH/4(lse) -> Mux14/4
  L BFSH/3(Vce) -> To Workspace105/1, Mux14/3
  L BFSH/2(Lce) -> To Workspace103/1, Mux14/2
  L BFSH/1(Fmtc) -> Mux14/1, Product18/1
  L BFSH/5(A) -> To Workspace104/1, Mux14/5
  L BFSH/6(fce [Fmax]) -> To Workspace106/1, Mux14/6
  Mux15/1 -> Terminator15/1
  L RF/1(Fmtc) -> Product19/2, Product20/2, Mux15/1
  L RF/2(Lce) -> To Workspace101/1, Mux15/2
  L RF/3(Vce) -> To Workspace98/1, Mux15/3
  L RF/4(lse) -> Mux15/4
  L RF/5(A) -> To Workspace96/1, Mux15/5
  L RF/6(fce [Fmax]) -> To Workspace99/1, Mux15/6
  L RF/7("fse [Fmax}") -> To Workspace100/1, Mux15/7
  L RF Link1/1(lmtu [m]) -> L RF/2(lmtu [m])
  [LBFSHstim] -> To Workspace102/1, L BFSH/1(STIM)
  L BFSH Link1/2(lever [m]) -> Product18/2
  Product18/1 -> Sum24/2
  Product2/1 -> Sum24/1, To Workspace94/1
  [LRFstim] -> To Workspace97/1, L RF/1(STIM)
  L RF Link1/3(lever23 [m]) -> Product20/1
  L RF Link1/2(lever34 [m]) -> Product19/1
  Product7/1 -> Sum25/1
  Product20/1 -> Sum25/2
  Product8/1 -> Sum26/1
  Product19/1 -> Sum26/2
  L BFSH/7("fse [Fmax}") -> Mux14/7, To Workspace107/1
  Product21/1 -> Sum27/2
  [RBFSHstim] -> To Workspace108/1, R BFSH/1(STIM)
  R BFSH/3(Vce) -> To Workspace111/1, Mux16/3
  R BFSH/2(Lce) -> To Workspace109/1, Mux16/2
  R BFSH/4(lse) -> Mux16/4
  R BFSH/7("fse [Fmax}") -> Mux16/7, To Workspace113/1
  L BFSH Link2/2(lever [m]) -> Product21/2
  L BFSH Link2/1(lmtu [m]) -> R BFSH/2(lmtu [m])
  R BFSH/6(fce [Fmax]) -> To Workspace112/1, Mux16/6
  R BFSH/5(A) -> To Workspace110/1, Mux16/5
  Mux16/1 -> Terminator16/1
  R BFSH/1(Fmtc) -> Mux16/1, Product21/1
  Sum27/1 -> Sum19/1
  [RRFstim] -> To Workspace117/1, R RF/1(STIM)
  Product22/1 -> Sum29/2
  Product23/1 -> Sum28/2
  L RF Link2/3(lever23 [m]) -> Product23/1
  R RF/6(fce [Fmax]) -> To Workspace119/1, Mux17/6
  Demux6/1 -> R Hip Joint Limits/1(phi [rad]), L HFL Link2/1(phi34 [rad]), L GLU Link1/1(phi34 [rad]), L RF Link2/1(phi34 [rad]), L HAM Link1/1(phi34 [rad])
  L RF Link2/1(lmtu [m]) -> R RF/2(lmtu [m])
  R RF/7("fse [Fmax}") -> To Workspace114/1, Mux17/7
  R RF/2(Lce) -> To Workspace115/1, Mux17/2
  R RF/1(Fmtc) -> Product22/2, Product23/2, Mux17/1
  Mux17/1 -> Terminator17/1
  R RF/4(lse) -> Mux17/4
  R RF/3(Vce) -> To Workspace118/1, Mux17/3
  Demux7/1 -> L GAS Link2/1(phi23 [rad]), L VAS Link2/1(phi23 [rad]), L BFSH Link2/1(phi23 [rad]), L RF Link2/2(phi23 [rad]), L HAM Link1/2(phi23 [rad]), R Knee Joint Limits/1(phi [rad])
  R RF/5(A) -> To Workspace116/1, Mux17/5
  L RF Link2/2(lever34 [m]) -> Product22/1
  Product16/1 -> Sum28/1
  Product17/1 -> Sum29/1
